simulink model "hfi_flux_pmsm"  (R2026a)
settings: Solver=FixedStepDiscrete  StartTime=0  StopTime=8.0  FixedStep=1/15000
PreLoadFcn:
  | addpath('F:\code\foc\Doc\matlab');
StartFcn:
  | clear sl_hfi_flux sl_hfi sl_flux sl_pmsm_discrete;
Description:
  | 闭环：VESC 风格按 ERPM 回差选择 HFI/Ortega 磁链角
settings Model: Creator=15403  LastModifiedBy=15403

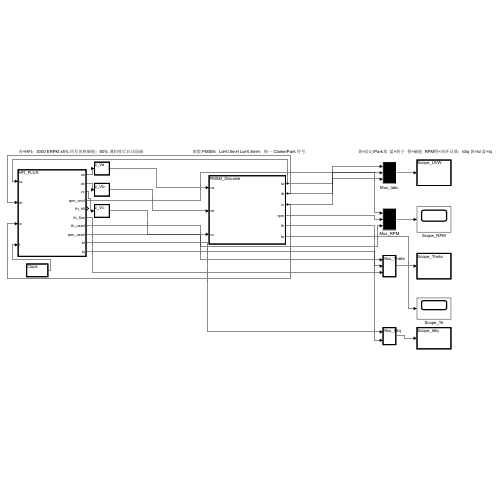
[thumbnail: Simulink's stored preview of the top-level diagram]
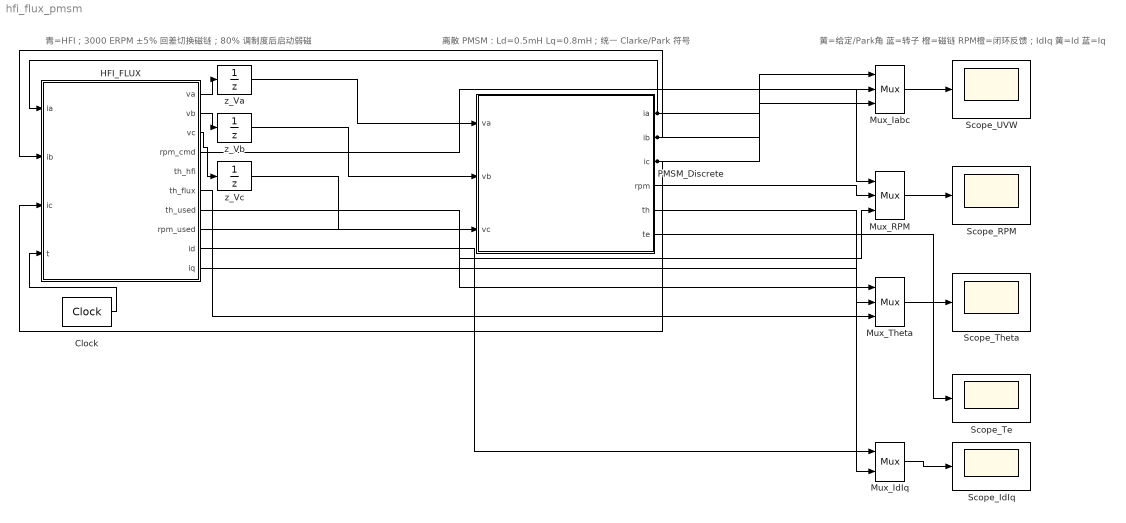
== system hfi_flux_pmsm ==
  note: 离散 PMSM：Ld=0.5mH Lq=0.8mH；统一 Clarke/Park 符号
  note: 黄=给定/Park角 蓝=转子 橙=磁链 RPM橙=闭环反馈；IdIq 黄=Id 蓝=Iq
  note: 青=HFI；3000 ERPM ±5% 回差切换磁链；80% 调制度后启动弱磁
  Clock : DigitalClock  SampleTime=1/15000
  HFI_FLUX : MATLAB Function  TreatAsAtomicUnit=on
  Mux_Iabc : Mux  Inputs=3
  Mux_IdIq : Mux  Inputs=2
  Mux_RPM : Mux  Inputs=3
  Mux_Theta : Mux  Inputs=3
  PMSM_Discrete : MATLAB Function  TreatAsAtomicUnit=on
  Scope_IdIq : Scope
  Scope_RPM : Scope
  Scope_Te : Scope
  Scope_Theta : Scope
  Scope_UVW : Scope
  z_Va : UnitDelay  SampleTime=1/15000
  z_Vb : UnitDelay  SampleTime=1/15000
  z_Vc : UnitDelay  SampleTime=1/15000
  wires:
  Clock/1 -> HFI_FLUX/4(t)
  HFI_FLUX/1(va) -> z_Va/1
  HFI_FLUX/2(vb) -> z_Vb/1
  HFI_FLUX/3(vc) -> z_Vc/1
  z_Va/1 -> PMSM_Discrete/1(va)
  z_Vb/1 -> PMSM_Discrete/2(vb)
  z_Vc/1 -> PMSM_Discrete/3(vc)
  PMSM_Discrete/1(ia) -> HFI_FLUX/1(ia), Mux_Iabc/1
  PMSM_Discrete/2(ib) -> HFI_FLUX/2(ib), Mux_Iabc/2
  PMSM_Discrete/3(ic) -> HFI_FLUX/3(ic), Mux_Iabc/3
  HFI_FLUX/4(rpm_cmd) -> Mux_RPM/1
  PMSM_Discrete/4(rpm) -> Mux_RPM/2
  HFI_FLUX/8(rpm_used) -> Mux_RPM/3
  HFI_FLUX/7(th_used) -> Mux_Theta/1
  PMSM_Discrete/5(th) -> Mux_Theta/2
  HFI_FLUX/6(th_flux) -> Mux_Theta/3
  Mux_Iabc/1 -> Scope_UVW/1
  Mux_RPM/1 -> Scope_RPM/1
  Mux_Theta/1 -> Scope_Theta/1
  PMSM_Discrete/6(te) -> Scope_Te/1
  HFI_FLUX/9(id) -> Mux_IdIq/1
  HFI_FLUX/10(iq) -> Mux_IdIq/2
  Mux_IdIq/1 -> Scope_IdIq/1

== matlab function hfi_flux_pmsm/PMSM_Discrete ==
  data: va input; ia output; vb input; vc input; ib output; ic output; rpm output; th output; te output
function [ia,ib,ic,rpm,th,te] = fcn(va,vb,vc)
[ia,ib,ic,rpm,th,te] = sl_pmsm_discrete(va,vb,vc);
end

== matlab function hfi_flux_pmsm/HFI_FLUX ==
  data: ia input; va output; ib input; ic input; t input; vb output; vc output; rpm_cmd output; th_hfi output; th_flux output; th_used output; rpm_used output; id output; iq output
function [va,vb,vc,rpm_cmd,th_hfi,th_flux,th_used,rpm_used,id,iq] = fcn(ia,ib,ic,t)
[va,vb,vc,rpm_cmd,th_hfi,th_flux,th_used,rpm_used,id,iq] = sl_hfi_flux(ia,ib,ic,t);
end
